simulink model "modele_freinage_regeneratif_v7"  (R2024a)
settings: Solver=VariableStepAuto  StartTime=0.0  StopTime=40  RelTol=1e-3
undefined symbols (not defined in the file): sigbuilder_block
libraries: simulink x2
settings Model: Creator=HP  LastModifiedBy=HP

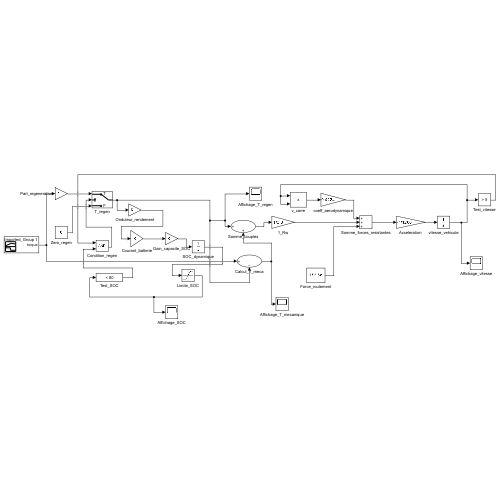
[thumbnail: Simulink's stored preview of the top-level diagram]
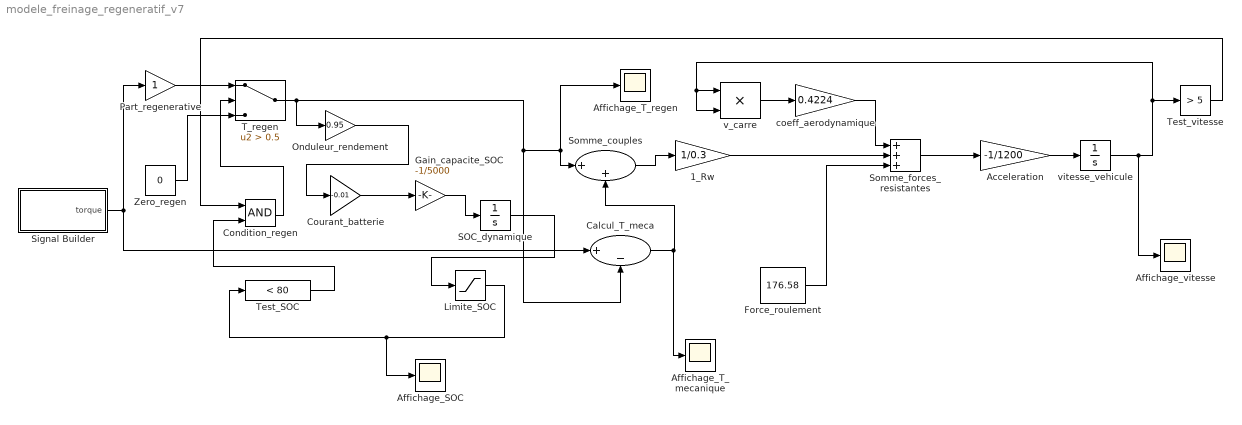
== system modele_freinage_regeneratif_v7 ==
  1_Rw : Gain  Gain=1/0.3
  "Acceleration " : Gain  Gain=-1/1200
  Affichage_SOC : Scope
  Affichage_T_mecanique : Scope
  Affichage_T_regen : Scope
  Affichage_vitesse : Scope
  Calcul_T_meca : Sum  Inputs=|+-
  Condition_regen : Logic  AllPortsSameDT=off  OutDataTypeStr=boolean
  Courant_batterie : Gain  Gain=-0.01
  Force_roulement : Constant  Value=176.58
  Gain_capacite_SOC : Gain  Gain=-1/5000
  Limite_SOC : Saturate  UpperLimit=100  LowerLimit=0
  Onduleur_rendement : Gain  Gain=0.95
  Part_regenerative : Gain
  SOC_dynamique : Integrator  InitialCondition=50
  Signal Builder : Subsystem  Tag=STV Subsys  LoadFcn=sigbuilder_block('load',[5.5 36 949 412 ]);  StartFcn=sigbuilder_block('start');  StopFcn=sigbuilder_block('stop');  ClipboardFcn=sigbuilder_block('clipboard');  mask(Sigbuilder block){tuvar=[0:10]}
      mask help: Simulink:masks:SigbuilderBlock_MD
      mask init:
      | if ~strcmp(get_param(bdroot(gcbh),'SimulationStatus'),'stopped') tuvar = sigbuilder_block('maskInit'); end
      settings: CopyFcn=sigbuilder_block('copy');  DeleteFcn=sigbuilder_block('delete');  ModelCloseFcn=sigbuilder_block('modelClose');  PreSaveFcn=sigbuilder_block('preSave');  PauseFcn=sigbuilder_block('pause');  ContinueFcn=sigbuilder_block('continue');  NameChangeFcn=sigbuilder_block('namechange');  OpenFcn=sigbuilder_block('open',[5.5 36 949 412 ]);  CloseFcn=sigbuilder_block('close');
      mask Display: plot(0, 0, 100, 100,[2, 2, 32, 32, 2], [68, 8, 8, 68, 68],[32, 2], [38, 38], [32, 19, 2],[53, 60, 44], [32, 17, 17, 2],[16, 16, 31, 31]);txt = getActiveGroup(gcbh);text(2, 100, txt,'verticalAlignment', 'top');
  Somme_couples : Sum  Inputs=|++
  Somme_forces_resistantes : Sum  Inputs=+++
  T_regen : Switch  Criteria=u2 > Threshold  Threshold=0.5  SaturateOnIntegerOverflow=off  InputSameDT=off
  Test_SOC : simulink/Logic and Bit Operations/Compare To Constant  relop=<  const=80  OutDataTypeStr=boolean
  Test_vitesse : simulink/Logic and Bit Operations/Compare To Constant  relop=>  const=5  OutDataTypeStr=boolean
  Zero_regen : Constant  Value=0
  coeff_aerodynamique : Gain  Gain=0.4224
  v_carre : Product
  vitesse_vehicule : Integrator  InitialCondition=50
  wires:
  Somme_forces_resistantes/1 -> "Acceleration "/1
  1_Rw/1 -> Somme_forces_resistantes/2
  v_carre/1 -> coeff_aerodynamique/1
  coeff_aerodynamique/1 -> Somme_forces_resistantes/1
  Force_roulement/1 -> Somme_forces_resistantes/3
  "Acceleration "/1 -> vitesse_vehicule/1
  vitesse_vehicule/1 -> Test_vitesse/1, v_carre/2, v_carre/1, Affichage_vitesse/1
  Signal Builder/1(torque) -> Part_regenerative/1, Calcul_T_meca/1
  Calcul_T_meca/1 -> Affichage_T_mecanique/1, Somme_couples/2
  Part_regenerative/1 -> T_regen/1
  Zero_regen/1 -> T_regen/3
  T_regen/1 -> Onduleur_rendement/1, Affichage_T_regen/1, Somme_couples/1, Calcul_T_meca/2
  Somme_couples/1 -> 1_Rw/1
  Test_SOC/1 -> Condition_regen/2
  Test_vitesse/1 -> Condition_regen/1
  Condition_regen/1 -> T_regen/2
  Courant_batterie/1 -> Gain_capacite_SOC/1
  Limite_SOC/1 -> Test_SOC/1, Affichage_SOC/1
  Gain_capacite_SOC/1 -> SOC_dynamique/1
  SOC_dynamique/1 -> Limite_SOC/1
  Onduleur_rendement/1 -> Courant_batterie/1

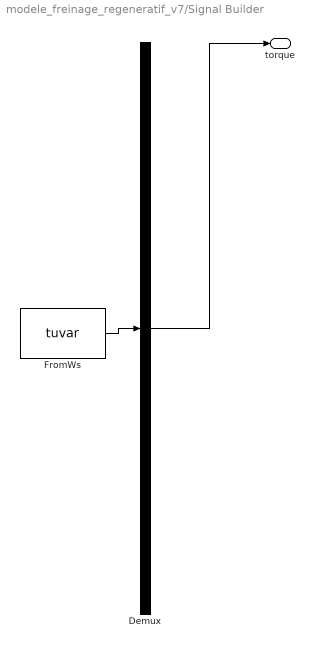
== system modele_freinage_regeneratif_v7/Signal Builder ==
  Demux : Demux  Tag=STV Demux  Outputs=1
      settings: DisplayOption=none
  FromWs : FromWorkspace  Tag=STV FromWs  VariableName=tuvar
      SigBuilderData=|
      | common.afterFinalStr = 'Extrapolate'
      | common.sampleTime = 0
      | dataSet(1).timeRange = [0 2.5]
      | dataSet(1).name = 'Imported_Group 1'
      | dataSet(2).timeRange = [0 2.5]
      | dataSet(2).name = 'Imported_Group 2'
      | sbobj.Name = 'Signal Builder'
      | sbobj.Groups(1).Name = 'Imported_Group 1'
      | sbobj.Groups(1).Signals.Name = 'torque'
      | sbobj.Groups(1).Signals.XData = [0 0.3 0.6 0.9 1.2 1.6 2 2.3 2.5]
      | sbobj.Groups(1).Signals.YData = [0 -100 -148 -150 -152 -150 -98 -47 0]
      | sbobj.Groups(1).TimeRange = [0 2.5]
      | sbobj.Groups(2).Name = 'Imported_Group 2'
      | sbobj.Groups(2).Signals.Name = 'torque'
      | sbobj.Groups(2).Signals.XData = [0 0.05 0.05 0.5 0.5 0.75 0.75 1.25 1.25 1.65 1.65 2.05 2.05 2.35 2.35 2.5]
      | sbobj.Groups(2).Signals.YData = [0 0 5 5 4 4 -1.4 -1.4 1.5 1.5 5 5 4 4 -1 -1]
      | sbobj.Groups(2).TimeRange = [0 2.5]
  torque : Outport  VectorParamsAs1DForOutWhenUnconnected=off
  wires:
  Demux/1 -> torque/1
  FromWs/1 -> Demux/1
